simulink model "simulation"  (R2020b)
settings: Solver=VariableStepAuto  StartTime=0.0  StopTime=10.0  RelTol=1e-3
values from neighbouring files (symbols this model uses):
  F2 = A2 - G2*C2    [Matlab_code.m]
  G2 = K_tild'    [Matlab_code.m]
  H2 = B2 - G2*D2    [Matlab_code.m]
  K2 = [K(1,1) K(1,2)]    [Matlab_code.m]
  Ki = -[K(1,3)]    [Matlab_code.m]
undefined symbols (not defined in the file or in its folder): A2x, B2x, C2x
settings Model: Creator=user  LastModifiedBy=user
settings DebuggingCC: UnconnectedInputMsg=none  UnconnectedOutputMsg=none  UnconnectedLineMsg=none
settings ModelReferenceCC: EnableRefExpFcnMdlSchedulingChecks=off
settings RTWCC: GPUComputeCapability=5.0
settings ConfigComp: CovBoundaryAbsTol=1.0e-5

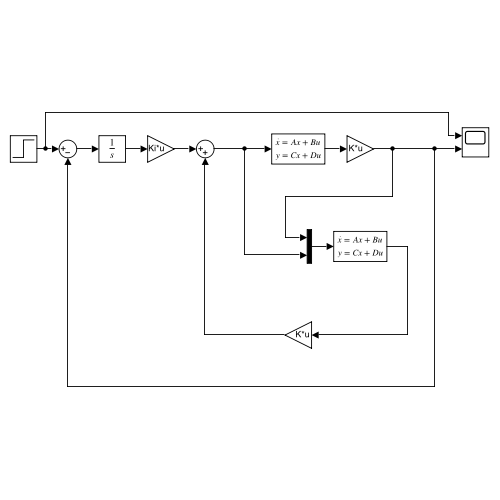
[thumbnail: Simulink's stored preview of the top-level diagram]
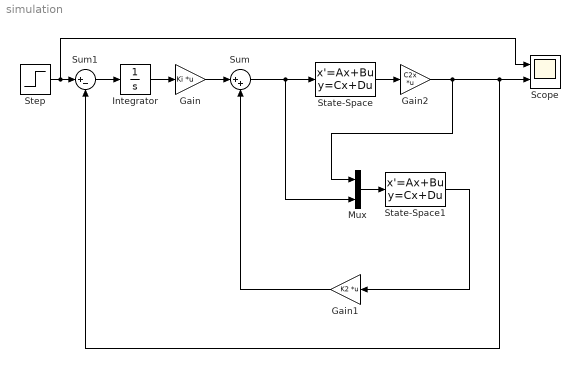
== system simulation ==
  Gain : Gain  Gain=Ki  Multiplication=Matrix(K*u)
  Gain1 : Gain  Gain=K2  Multiplication=Matrix(K*u)
  Gain2 : Gain  Gain=C2x  Multiplication=Matrix(K*u)
  Integrator : Integrator
  Mux : Mux  Inputs=2
  Scope : Scope  NumInputPorts=2
  State-Space : StateSpace  A=A2x  B=B2x  C=eye(2)  D=[0;0]  InitialCondition=0
  State-Space1 : StateSpace  A=F2  B=[G2 H2]  C=eye(2)  D=zeros(2,2)  InitialCondition=0
  Step : Step  SampleTime=0
  Sum : Sum  Inputs=|++
  Sum1 : Sum  Inputs=|+-
  wires:
  Integrator/1 -> Gain/1
  Gain/1 -> Sum/1
  Sum/1 -> Mux/2, State-Space/1
  State-Space1/1 -> Gain1/1
  Gain1/1 -> Sum/2
  Sum1/1 -> Integrator/1
  Mux/1 -> State-Space1/1
  State-Space/1 -> Gain2/1
  Gain2/1 -> Mux/1, Scope/2, Sum1/2
  Step/1 -> Scope/1, Sum1/1
